simulink model "uartReceDemo"  (R2023a)
settings: Solver=ode4  StartTime=0.0  StopTime=0.011  FixedStep=0.01  RelTol=1e-3
libraries: simulink x8, instrumentseriallib x3, svdutilitieslib x1, slrealtimeutilitieslib x1
settings Model: Creator=User  LastModifiedBy=zqinghua
settings SolverCC: AlgebraicLoopSolver=TrustRegion
settings DebuggingCC: ArithmeticOperatorsInVariantConditions=warning
settings SFSimCC: CustomCodeUndefinedFunction=UseInterfaceOnly
settings CodeAppCC: StateflowObjectComments=on

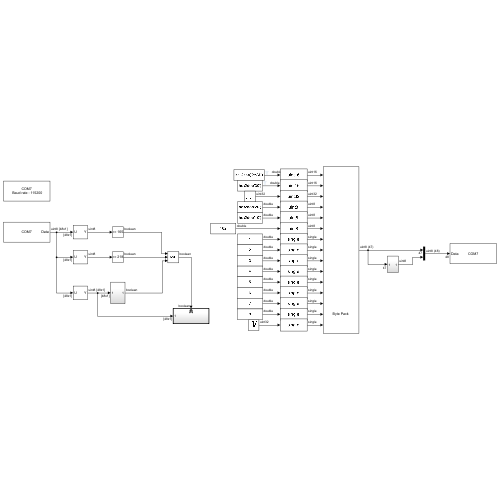
[thumbnail: Simulink's stored preview of the top-level diagram]
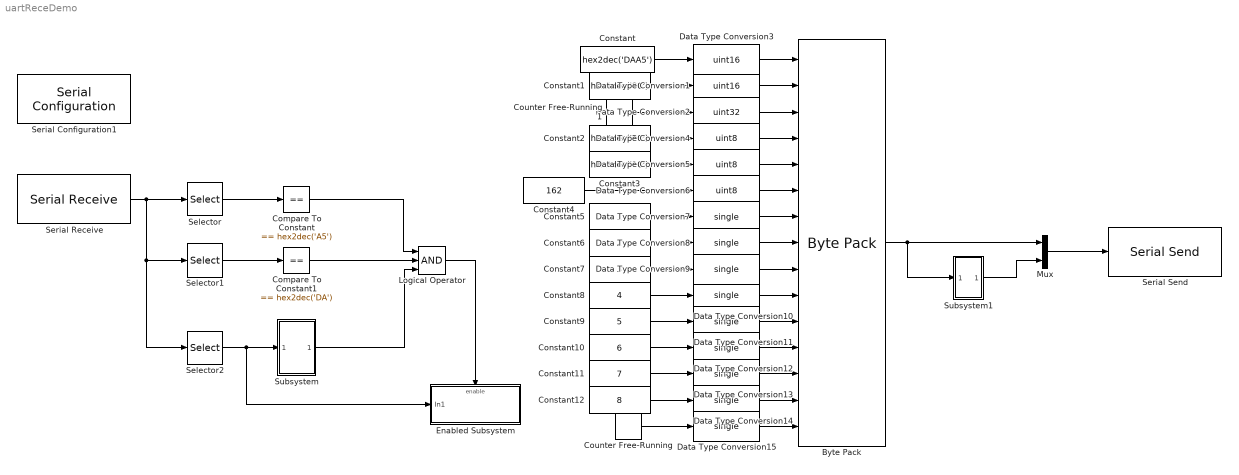
== system uartReceDemo ==
  Byte Pack : svdutilitieslib/Byte Pack  maskPackedDataType=uint8  datatypes={'uint16','uint16','uint32','uint8','uint8','uint8','single','single','single','single','single','single','single','single','single'}  byteAlign=1  blockPlatform=tic2000
      settings: LibrarySourceBlock=c2000lib/Target Communication/Byte Pack
  Compare To Constant : simulink/Logic and Bit Operations/Compare To Constant  relop===  const=hex2dec('A5')  OutDataTypeStr=boolean
  Compare To Constant1 : simulink/Logic and Bit Operations/Compare To Constant  relop===  const=hex2dec('DA')  OutDataTypeStr=boolean
  Constant : Constant  Value=hex2dec('DAA5')  SampleTime=-1
  Constant1 : Constant  Value=hex2dec('30')  SampleTime=-1
  Constant10 : Constant  Value=6  SampleTime=-1
  Constant11 : Constant  Value=7  SampleTime=-1
  Constant12 : Constant  Value=8  SampleTime=-1
  Constant2 : Constant  Value=hex2dec('20')  SampleTime=-1
  Constant3 : Constant  Value=hex2dec('10')  SampleTime=-1
  Constant4 : Constant  Value=162  SampleTime=-1
  Constant5 : Constant  SampleTime=-1
  Constant6 : Constant  Value=2  SampleTime=-1
  Constant7 : Constant  Value=3  SampleTime=-1
  Constant8 : Constant  Value=4  SampleTime=-1
  Constant9 : Constant  Value=5  SampleTime=-1
  Counter Free-Running : simulink/Sources/Counter Free-Running  NumBits=32  tsamp=-1
  Counter Free-Running1 : simulink/Sources/Counter Free-Running  NumBits=32  tsamp=-1
  Data Type Conversion1 : DataTypeConversion  OutDataTypeStr=uint16  SaturateOnIntegerOverflow=off  RndMeth=Floor
  Data Type Conversion{7..15} (9 alike) : DataTypeConversion  OutDataTypeStr=single  SaturateOnIntegerOverflow=off  RndMeth=Floor
  Data Type Conversion2 : DataTypeConversion  OutDataTypeStr=uint32  SaturateOnIntegerOverflow=off  RndMeth=Floor
  Data Type Conversion3 : DataTypeConversion  OutDataTypeStr=uint16  SaturateOnIntegerOverflow=off  RndMeth=Floor
  Data Type Conversion4 : DataTypeConversion  OutDataTypeStr=uint8  SaturateOnIntegerOverflow=off  RndMeth=Floor
  Data Type Conversion5 : DataTypeConversion  OutDataTypeStr=uint8  SaturateOnIntegerOverflow=off  RndMeth=Floor
  Data Type Conversion6 : DataTypeConversion  OutDataTypeStr=uint8  SaturateOnIntegerOverflow=off  RndMeth=Floor
  Enabled Subsystem : Subsystem  TreatAsAtomicUnit=on
  Logical Operator : Logic  Inputs=3  AllPortsSameDT=off  OutDataTypeStr=boolean
  Mux : Mux  Inputs=2
  Selector : Selector  InputPortWidth=48  IndexOptions=Index vector (dialog)  Indices=[1]  OutputSizes=1
  Selector1 : Selector  InputPortWidth=48  IndexOptions=Index vector (dialog)  Indices=[2]  OutputSizes=1
  Selector2 : Selector  InputPortWidth=48  IndexOptions=Index vector (dialog)  Indices=[1:48]  OutputSizes=1
  Serial Configuration1 : instrumentseriallib/Serial Configuration  Priority=-200000  PortSel=COM7  Port=COM7  ComPort=COM7  BaudRate=115200  DataBits=8  Parity=none  StopBits=1  ByteOrder=little-endian  FlowControl=none  Timeout=10  SimulateUsing=Interpreted execution  BlockInModel=on  aMode=1
  Serial Receive : instrumentseriallib/Serial Receive  Priority=1  PortSel=COM7  Port=COM7  ComPort=COM7  DataType=uint8  SaveDataType=uint8  ToggleHeader=off  Header=[]  ToggleTerminator=on  Terminator=<none>  CustomTerminator=[]  InputFormat=Column major  ToggleDataSize=on  DataSize=48  EnableBlockingMode=on  ActionDataUnavailable=Output last received value  ActionWhenDataUnavailable=Output last received value  CustomValue=0  SampleTime=-1  SimulateUsing=Interpreted execution  BlockInModel=on  aMode=1
  Serial Send : instrumentseriallib/Serial Send  Priority=1  PortSel=COM7  Port=COM7  ComPort=COM7  Header=[]  Terminator=<none>  CustomTerminator=[]  EnableBlockingMode=on  SimulateUsing=Interpreted execution  BlockInModel=on  aMode=1
  Subsystem : Subsystem
  Subsystem1 : Subsystem
  wires:
  Serial Receive/1 -> Selector/1, Selector1/1, Selector2/1
  Selector/1 -> Compare To Constant/1
  Selector1/1 -> Compare To Constant1/1
  Compare To Constant/1 -> Logical Operator/1
  Compare To Constant1/1 -> Logical Operator/2
  Selector2/1 -> Enabled Subsystem/1(In1), Subsystem/1(In1)
  Logical Operator/1 -> Enabled Subsystem/Enable
  Subsystem/1(Out1) -> Logical Operator/3
  Data Type Conversion4/1 -> Byte Pack/4
  Data Type Conversion5/1 -> Byte Pack/5
  Data Type Conversion8/1 -> Byte Pack/8
  Data Type Conversion3/1 -> Byte Pack/1
  Constant5/1 -> Data Type Conversion7/1
  Constant8/1 -> Data Type Conversion10/1
  Constant6/1 -> Data Type Conversion8/1
  Data Type Conversion11/1 -> Byte Pack/11
  Constant11/1 -> Data Type Conversion13/1
  Data Type Conversion10/1 -> Byte Pack/10
  Constant10/1 -> Data Type Conversion12/1
  Constant7/1 -> Data Type Conversion9/1
  Data Type Conversion7/1 -> Byte Pack/7
  Constant2/1 -> Data Type Conversion4/1
  Counter Free-Running1/1 -> Data Type Conversion2/1
  Mux/1 -> Serial Send/1
  Data Type Conversion2/1 -> Byte Pack/3
  Counter Free-Running/1 -> Data Type Conversion15/1
  Data Type Conversion13/1 -> Byte Pack/13
  Data Type Conversion6/1 -> Byte Pack/6
  Data Type Conversion9/1 -> Byte Pack/9
  Constant/1 -> Data Type Conversion3/1
  Constant12/1 -> Data Type Conversion14/1
  Constant9/1 -> Data Type Conversion11/1
  Subsystem1/1(Out1) -> Mux/2
  Data Type Conversion12/1 -> Byte Pack/12
  Constant4/1 -> Data Type Conversion6/1
  Data Type Conversion15/1 -> Byte Pack/15
  Constant1/1 -> Data Type Conversion1/1
  Constant3/1 -> Data Type Conversion5/1
  Data Type Conversion14/1 -> Byte Pack/14
  Byte Pack/1 -> Subsystem1/1(In1), Mux/1
  Data Type Conversion1/1 -> Byte Pack/2

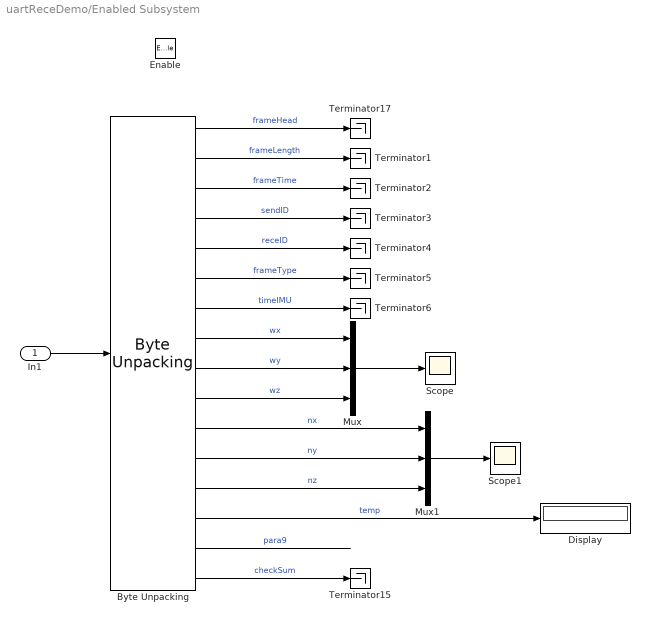
== system uartReceDemo/Enabled Subsystem ==
  In1 : Inport
  Enable : EnablePort
  "Byte Unpacking " : slrealtimeutilitieslib/Byte Unpacking  MaskUnpackedDataTypes={'uint16','uint16','uint32','uint8','uint8','uint8','single','single','single','single','single','single','single','single','single','uint8'}  MaskUnpackedDataSizes={1,1,1,1,1,1,1,1,1,1,1,1,1,1,1,1}  MaskAlignment=1
  Display : Display
  Mux : Mux  Inputs=3
  Mux1 : Mux  Inputs=3
  Scope : Scope
  Scope1 : Scope
  Terminator{1..6,15,17} (8 alike) : Terminator
  wires:
  "Byte Unpacking "/11 -> Mux1/1  "nx"
  "Byte Unpacking "/1 -> Terminator17/1  "frameHead"
  "Byte Unpacking "/8 -> Mux/1  "wx"
  "Byte Unpacking "/13 -> Mux1/3  "nz"
  "Byte Unpacking "/5 -> Terminator4/1  "receID"
  "Byte Unpacking "/14 -> Display/1  "temp"
  "Byte Unpacking "/6 -> Terminator5/1  "frameType"
  "Byte Unpacking "/3 -> Terminator2/1  "frameTime"
  "Byte Unpacking "/2 -> Terminator1/1  "frameLength"
  "Byte Unpacking "/16 -> Terminator15/1  "checkSum"
  "Byte Unpacking "/15 -> ?  "para9"
  "Byte Unpacking "/12 -> Mux1/2  "ny"
  "Byte Unpacking "/10 -> Mux/3  "wz"
  "Byte Unpacking "/9 -> Mux/2  "wy"
  "Byte Unpacking "/7 -> Terminator6/1  "timeIMU"
  "Byte Unpacking "/4 -> Terminator3/1  "sendID"
  In1/1 -> "Byte Unpacking "/1
  Mux/1 -> Scope/1
  Mux1/1 -> Scope1/1

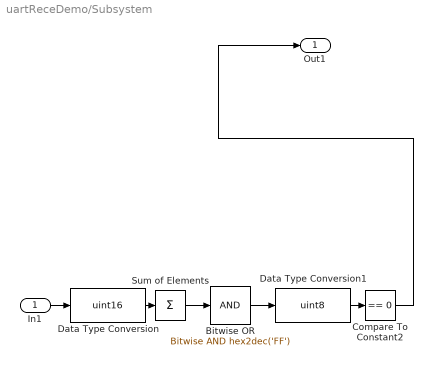
== system uartReceDemo/Subsystem ==
  In1 : Inport
  Bitwise OR : simulink/Logic and Bit Operations/Bitwise Operator  logicop=AND  UseBitMask=on  BitMask=hex2dec('FF')  BitMaskRealWorld=Stored Integer
  Compare To Constant2 : simulink/Logic and Bit Operations/Compare To Constant  relop===  const=0  OutDataTypeStr=boolean
  Data Type Conversion : DataTypeConversion  OutDataTypeStr=uint16  SaturateOnIntegerOverflow=off  RndMeth=Floor
  Data Type Conversion1 : DataTypeConversion  OutDataTypeStr=uint8  SaturateOnIntegerOverflow=off  RndMeth=Floor
  Sum of Elements : Sum  Inputs=+
  Out1 : Outport
  wires:
  Compare To Constant2/1 -> Out1/1
  Sum of Elements/1 -> Bitwise OR/1
  Bitwise OR/1 -> Data Type Conversion1/1
  Data Type Conversion/1 -> Sum of Elements/1
  Data Type Conversion1/1 -> Compare To Constant2/1
  In1/1 -> Data Type Conversion/1

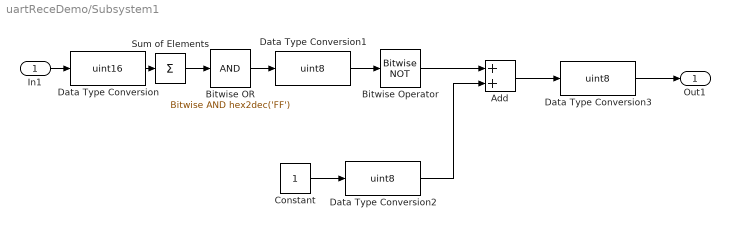
== system uartReceDemo/Subsystem1 ==
  In1 : Inport
  Add : Sum
  Bitwise Operator : simulink/Logic and Bit Operations/Bitwise Operator  logicop=NOT  UseBitMask=off  BitMask=bin2dec('11011001')  BitMaskRealWorld=Stored Integer
  Bitwise OR : simulink/Logic and Bit Operations/Bitwise Operator  logicop=AND  UseBitMask=on  BitMask=hex2dec('FF')  BitMaskRealWorld=Stored Integer
  Constant : Constant
  Data Type Conversion : DataTypeConversion  OutDataTypeStr=uint16  SaturateOnIntegerOverflow=off  RndMeth=Floor
  Data Type Conversion1 : DataTypeConversion  OutDataTypeStr=uint8  SaturateOnIntegerOverflow=off  RndMeth=Floor
  Data Type Conversion2 : DataTypeConversion  OutDataTypeStr=uint8  SaturateOnIntegerOverflow=off  RndMeth=Floor
  Data Type Conversion3 : DataTypeConversion  OutDataTypeStr=uint8  SaturateOnIntegerOverflow=off  RndMeth=Floor
  Sum of Elements : Sum  Inputs=+
  Out1 : Outport
  wires:
  Data Type Conversion3/1 -> Out1/1
  Sum of Elements/1 -> Bitwise OR/1
  Bitwise OR/1 -> Data Type Conversion1/1
  Data Type Conversion/1 -> Sum of Elements/1
  Data Type Conversion1/1 -> Bitwise Operator/1
  In1/1 -> Data Type Conversion/1
  Bitwise Operator/1 -> Add/1
  Constant/1 -> Data Type Conversion2/1
  Data Type Conversion2/1 -> Add/2
  Add/1 -> Data Type Conversion3/1
